simulink model "arducopter"  (R2024b)
settings: Solver=FixedStepAuto  StartTime=0.0  StopTime=simIn.param.timeEnd  FixedStep=simIn.param.dt  RelTol=1e-3
undefined symbols (not defined in the file or in its folder): DiscIntNeverNeededParam, sim, simIn
libraries: simulink x60, slident x4, vrlib x1
(part 7 of 9)

== system arducopter/Attitude Controller/input_euler_angle_roll_pitch_euler_rate_yaw()/Feedforward enabled/input shaping/input shaping yaw rate ==
  note: AC_AttitudeControl::input_shaping_ang_vel()
      | Limits the maximum acceleration resulting from the target yaw rate, so that the target yaw rate is slewed towards the input rate
  yawRateDes : Inport
  yawRateTar : Inport  Port=2
  eulerAccelMax : Inport  Port=3
  Constant2 : Constant  Value=simIn.param.dt  VectorParams1D=off
  Constant3 : Constant  Value=simIn.param.PILOT_Y_RATE_TC  VectorParams1D=off
  Data Type Conversion1 : DataTypeConversion  OutDataTypeStr=single  SaturateOnIntegerOverflow=off  RndMeth=Floor
  MATLAB Function1 : MATLAB Function  TreatAsAtomicUnit=on
  Square Root Controller : Subsystem  TreatAsAtomicUnit=on
  eulerYawRateTar : Outport
  wires:
  yawRateDes/1 -> MATLAB Function1/1(desiredAngVel)
  eulerAccelMax/1 -> MATLAB Function1/3(accelMax)
  MATLAB Function1/1(eulerRateTar) -> eulerYawRateTar/1
  yawRateTar/1 -> MATLAB Function1/2(targetAngVel)
  Data Type Conversion1/1 -> MATLAB Function1/4(dt)
  Constant2/1 -> Data Type Conversion1/1
  Constant3/1 -> MATLAB Function1/5(input_tc)

== system arducopter/Attitude Controller/input_euler_angle_roll_pitch_euler_rate_yaw()/thrust_heading_rotation_angles()/Yaw error limitation/Second limiting condition  ==
  note: Output adapted attitudeTarget and attitudeError if yaw limiting condition is met. Otherwise output old values.
  note: Second limiting condition: if (!is_zero(_p_angle_yaw.kP()) && fabsf(attitude_error.z) > heading_error_max)
  attitudeErrorIn : Inport
  attitudeTargetIn : Inport  Port=2
  thrustVecCorrection : Inport  Port=3
  attitudeBody : Inport  Port=4
  Enable : EnablePort
  Abs : Abs  SaturateOnIntegerOverflow=off
  Compare To Zero : simulink/Logic and Bit Operations/Compare To Zero  relop=~=  OutDataTypeStr=boolean
  Constant3 : Constant  Value=simIn.param.ATC.ACCEL_Y_CONTROLLER_MAX_RADSS
  Constant4 : Constant  Value=simIn.param.ATC.ACCEL_Y_CONTROLLER_MIN_RADSS
  Constant5 : Constant  Value=1/simIn.param.PIDY.P
  Constant6 : Constant  Value=simIn.param.ATC.ACCEL_Y_MAX
  Constant7 : Constant  Value=simIn.param.ATC.ANG_YAW_P
  Constant8 : Constant  Value=simIn.param.ATC.YAW_MAX_ERROR_ANGLE
  Gain1 : Gain  Gain=0.5
  Inverse Square Root Controller : MATLAB Function  TreatAsAtomicUnit=on
  Logical Operator : Logic  AllPortsSameDT=off  OutDataTypeStr=boolean
  Max : MinMax  Function=max  Inputs=2
  Min : MinMax  Inputs=2
  Min1 : MinMax  Inputs=2
  Relational Operator : RelationalOperator  Operator=>  OutDataTypeStr=boolean  RndMeth=Simplest  InputSameDT=off
  Selector2 : Selector  InputPortWidth=3  IndexOptions=Index vector (dialog)  Indices=[3]  OutputSizes=1
  Switch : Switch  Criteria=u2 > Threshold  SaturateOnIntegerOverflow=off  InputSameDT=off
  Switch1 : Switch  Criteria=u2 > Threshold  SaturateOnIntegerOverflow=off  InputSameDT=off
  Yaw limiting and recalculation of attitudeTarget : Subsystem
  attitudeTarget : Outport
  attitudeError : Outport  Port=2
  wires:
  attitudeErrorIn/1 -> [attitudeError]
  Max/1 -> Min/1
  Gain1/1 -> Max/1
  Constant3/1 -> Min/2
  Constant6/1 -> Gain1/1
  Constant4/1 -> Max/2
  Constant5/1 -> Inverse Square Root Controller/1(output)
  Constant7/1 -> Compare To Zero/1, Inverse Square Root Controller/2(p)
  Min/1 -> Inverse Square Root Controller/3(D_max)  "heading_accel_max"
  Constant8/1 -> Min1/2
  Inverse Square Root Controller/1(error) -> Min1/1
  Min1/1 -> Yaw limiting and recalculation of attitudeTarget/2(heading_error_max), Relational Operator/2  "heading_error_max"
  [attitudeError] -> Selector2/1
  Selector2/1 -> Abs/1
  Relational Operator/1 -> Logical Operator/2
  Compare To Zero/1 -> Logical Operator/1
  Abs/1 -> Relational Operator/1
  [attitudeError] -> Switch1/3
  Switch1/1 -> attitudeError/1
  Yaw limiting and recalculation of attitudeTarget/1(attitudeTarget) -> Switch/1
  [attitudeTarget] -> Switch/3
  Yaw limiting and recalculation of attitudeTarget/2(attitudeError) -> Switch1/1
  Switch/1 -> attitudeTarget/1
  Logical Operator/1 -> Yaw limiting and recalculation of attitudeTarget/Enable, Switch1/2, Switch/2
  attitudeBody/1 -> Yaw limiting and recalculation of attitudeTarget/4(attitudeBody)
  thrustVecCorrection/1 -> Yaw limiting and recalculation of attitudeTarget/3(thrustVecCorrection)
  [attitudeError] -> Yaw limiting and recalculation of attitudeTarget/1(attitudeErrorIn)
  attitudeTargetIn/1 -> [attitudeTarget]

== system arducopter/Attitude Controller/input_euler_angle_roll_pitch_euler_rate_yaw()/Feedforward enabled/input shaping/input shaping pitch angle/Square Root Controller1 ==
  sqrt_controller : TriggerPort  TriggerType=function-call  IsSimulinkFunction=on  FunctionName=sqrt_controller  FunctionVisibility=scoped  VariantControl=(inherit)
  Square Root Controller : MATLAB Function  TreatAsAtomicUnit=on
  output : ArgIn  DisableCoverage=on  OutDataTypeStr=single  ArgumentName=err
  p : ArgIn  DisableCoverage=on  Port=2  OutDataTypeStr=single  ArgumentName=p
  D_max : ArgIn  DisableCoverage=on  Port=3  OutDataTypeStr=single  ArgumentName=second_ord_lim
  output1 : ArgIn  DisableCoverage=on  Port=4  OutDataTypeStr=single  ArgumentName=dt
  correctionRate : ArgOut  DisableCoverage=on  OutDataTypeStr=single  ArgumentName=correctionRate
  wires:
  output/1 -> Square Root Controller/1(err)
  p/1 -> Square Root Controller/2(p)
  D_max/1 -> Square Root Controller/3(second_ord_lim)
  Square Root Controller/1(correction_rate) -> correctionRate/1
  output1/1 -> Square Root Controller/4(dt)

== system arducopter/Attitude Controller/input_euler_angle_roll_pitch_euler_rate_yaw()/Feedforward enabled/input shaping/input shaping pitch angle/calc p from input_tc ==
  note: Calculation of proportional factor of square root controller.
      | Based on function argument of sqrt_controller() in AC_AttitudeControl::input_shaping_angle()
  input_tc : Inport
  Constant2 : Constant  Value=0.01  OutDataTypeStr=single
  Constant3 : Constant  OutDataTypeStr=single
  Divide : Product  Inputs=*/
  Max : MinMax  Function=max  Inputs=2
  p : Outport
  wires:
  Constant2/1 -> Max/2
  Max/1 -> Divide/2
  Constant3/1 -> Divide/1
  input_tc/1 -> Max/1
  Divide/1 -> p/1

== system arducopter/Attitude Controller/input_euler_angle_roll_pitch_euler_rate_yaw()/Feedforward enabled/input shaping/input shaping roll angle/Square Root Controller1 ==
  sqrt_controller : TriggerPort  TriggerType=function-call  IsSimulinkFunction=on  FunctionName=sqrt_controller  FunctionVisibility=scoped  VariantControl=(inherit)
  Square Root Controller : MATLAB Function  TreatAsAtomicUnit=on
  output : ArgIn  DisableCoverage=on  OutDataTypeStr=single  ArgumentName=err
  p : ArgIn  DisableCoverage=on  Port=2  OutDataTypeStr=single  ArgumentName=p
  D_max : ArgIn  DisableCoverage=on  Port=3  OutDataTypeStr=single  ArgumentName=second_ord_lim
  output1 : ArgIn  DisableCoverage=on  Port=4  OutDataTypeStr=single  ArgumentName=dt
  correctionRate : ArgOut  DisableCoverage=on  OutDataTypeStr=single  ArgumentName=correctionRate
  wires:
  output/1 -> Square Root Controller/1(err)
  p/1 -> Square Root Controller/2(p)
  D_max/1 -> Square Root Controller/3(second_ord_lim)
  Square Root Controller/1(correction_rate) -> correctionRate/1
  output1/1 -> Square Root Controller/4(dt)

== system arducopter/Attitude Controller/input_euler_angle_roll_pitch_euler_rate_yaw()/Feedforward enabled/input shaping/input shaping roll angle/calc p from input_tc ==
  note: Calculation of proportional factor of square root controller.
      | Based on function argument of sqrt_controller() in AC_AttitudeControl::input_shaping_angle()
  input_tc : Inport
  Constant2 : Constant  Value=0.01  OutDataTypeStr=single
  Constant3 : Constant  OutDataTypeStr=single
  Divide : Product  Inputs=*/
  Max : MinMax  Function=max  Inputs=2
  p : Outport
  wires:
  Constant2/1 -> Max/2
  Max/1 -> Divide/2
  Constant3/1 -> Divide/1
  input_tc/1 -> Max/1
  Divide/1 -> p/1

== system arducopter/Attitude Controller/input_euler_angle_roll_pitch_euler_rate_yaw()/Feedforward enabled/input shaping/input shaping yaw rate/Square Root Controller ==
  sqrt_controller : TriggerPort  TriggerType=function-call  IsSimulinkFunction=on  FunctionName=sqrt_controller  FunctionVisibility=scoped  VariantControl=(inherit)
  Square Root Controller : MATLAB Function  TreatAsAtomicUnit=on
  output : ArgIn  DisableCoverage=on  OutDataTypeStr=single  ArgumentName=err
  p : ArgIn  DisableCoverage=on  Port=2  OutDataTypeStr=single  ArgumentName=p
  D_max : ArgIn  DisableCoverage=on  Port=3  OutDataTypeStr=single  ArgumentName=second_ord_lim
  output1 : ArgIn  DisableCoverage=on  Port=4  OutDataTypeStr=single  ArgumentName=dt
  correctionRate : ArgOut  DisableCoverage=on  OutDataTypeStr=single  ArgumentName=correctionRate
  wires:
  output/1 -> Square Root Controller/1(err)
  p/1 -> Square Root Controller/2(p)
  D_max/1 -> Square Root Controller/3(second_ord_lim)
  Square Root Controller/1(correction_rate) -> correctionRate/1
  output1/1 -> Square Root Controller/4(dt)

== system arducopter/Attitude Controller/input_euler_angle_roll_pitch_euler_rate_yaw()/thrust_heading_rotation_angles()/Yaw error limitation/Second limiting condition /Yaw limiting and recalculation of attitudeTarget ==
  note: Limitation of yaw error
  note: Create new attitudeError with limited yaw error
  note: Calculate new attitudeTarget with limited headingVecCorrection
  attitudeErrorIn : Inport
  heading_error_max : Inport  Port=2
  thrustVecCorrection : Inport  Port=3
  attitudeBody : Inport  Port=4
  Enable : EnablePort
  Constant2 : Constant  Value=0  OutDataTypeStr=single
  Demux : Demux  Outputs=2
  Gain : Gain  Gain=-1
  MATLAB Function1 : MATLAB Function  TreatAsAtomicUnit=on
  MATLAB Function2 : MATLAB Function  TreatAsAtomicUnit=on
  MATLAB Function5 : MATLAB Function  TreatAsAtomicUnit=on
  MATLAB Function9 : MATLAB Function  TreatAsAtomicUnit=on
  Max : MinMax  Function=max  Inputs=2
  Min : MinMax  Inputs=2
  Mux : Mux  Inputs=3
  Mux1 : Mux  Inputs=3
  Selector : Selector  InputPortWidth=3  IndexOptions=Index vector (dialog)  Indices=[3]  OutputSizes=1
  Selector1 : Selector  InputPortWidth=3  IndexOptions=Index vector (dialog)  Indices=[1 2]  OutputSizes=1
  attitudeTarget : Outport
  attitudeError : Outport  Port=2
  wires:
  attitudeErrorIn/1 -> [attitudeError]
  Mux/1 -> MATLAB Function5/1(vec)
  MATLAB Function1/1(qRes) -> attitudeTarget/1
  MATLAB Function9/1(qRes) -> MATLAB Function1/2(q2)
  Min/1 -> Mux1/3, Mux/3
  Mux1/1 -> attitudeError/1
  Selector1/1 -> Demux/1
  Constant2/1 -> Mux/2, Mux/1
  [attitudeError] -> Selector1/1
  attitudeBody/1 -> MATLAB Function1/1(q1)
  Demux/2 -> Mux1/2
  Demux/1 -> Mux1/1
  thrustVecCorrection/1 -> MATLAB Function9/1(q1)
  MATLAB Function5/1(q) -> MATLAB Function9/2(q2)  "headingVecCorrection"
  heading_error_max/1 -> Min/2, Gain/1
  [attitudeError] -> Selector/1
  Gain/1 -> Max/2
  MATLAB Function2/1(radLim) -> Max/1
  Max/1 -> Min/1
  Selector/1 -> MATLAB Function2/1(radIn)

== matlab function arducopter/Position Controller/set_pos_target_z_from_climb_rate()/input_vel_accel_z/MATLAB Function ==
  data: overspeedGain output; velMaxUp input; velMaxDn input; velDes input; overspeedGainDefault input
function overspeedGain = calcOverspeedGain(velMaxUp, velMaxDn, velDes, overspeedGainDefault)
% Calculate increased maximum acceleration and jerk if over speed condition
% is detected
% Code based on AC_PosControl::calculate_overspeed_gain()
overspeedGain = single(1);
if velDes < velMaxDn && velMaxDn ~= 0
    overspeedGain = overspeedGainDefault * velDes / velMaxDn;
end
if velDes > velMaxUp && velMaxUp ~= 0
    overspeedGain = overspeedGainDefault * velDes / velMaxUp;
end

== matlab function arducopter/Position Controller/set_pos_target_z_from_climb_rate()/input_vel_accel_z/update_pos_vel_accel/MATLAB Function ==
  data: posIn input; pos output; velIn input; accIn input; dt input; limit input; vel output; posErr input; velErr input
function [pos, vel] = updatePosVelAccel(posIn, velIn, accIn, dt, limit, posErr, velErr)
% Single axis projection of position and velocity forwards in time based on
% a time step of dt and acceleration off acc.
% Based on update_pos_vel_accel() in control.cpp

% Move position and velocity forward by dt if it does not increase error
% when limited
deltaPos = velIn * dt + accIn * 0.5 * dt^2;
% do not add delta_pos if it will increase the velocity error in the direction of limit
if ((deltaPos * limit) > 0 && (posErr * limit) > 0)
    deltaPos = single(0);
end

pos = posIn + deltaPos;

% The next lines are based on update_vel_accel() which is called from
% update_pos_vel_accel()
deltaVel = accIn * dt;
% do not add delta_vel if it will increase the velocity error in the direction of limit
if ((deltaVel * limit) > 0 && (velErr * limit) > 0)
    if ((velIn * limit) < 0)
        deltaVel = min(max(deltaVel, -abs(velIn)), abs(velIn));
    else
        deltaVel = single(0);
    end
end
vel = velIn + deltaVel;

== matlab function arducopter/Position Controller/set z component of limit vec/MATLAB Function ==
  data: limLower input; limVecZ output; limUpper input
function limVecZ = fcn(limLower, limUpper)
% Based on AC_PosControl::update_z_controller()

if limUpper
    limVecZ = single(1);
elseif limLower
    limVecZ = single(-1);
else
    limVecZ = single(0);
end

== matlab function arducopter/Position Controller/set_pos_target_z_from_climb_rate()/input_vel_accel_z/shape_vel_accel/calc_KPa ==
  data: velErr output; velIn input; KPa output; vel input; accMin input; accMax input; jerkMax input
function [velErr, KPa] = calcKPa(velIn, vel, accMin, accMax, jerkMax)
% First part of shape_vel_accel() in control.cpp
% Calculates correction gain KPa for the square root controller based on
% the jerk and acceleration limits.

% Velocity error to be corrected
velErr = velIn - vel;

% Calculate time constants and limits to ensure stable operation.
% The direction of acceleration limit is the same as the velocity error.
% This is because the velocity error is negative when slowing down while
% closing a positive position error.
if velErr > 0
    KPa = jerkMax / accMax;
else
    KPa = jerkMax / (-accMin);
end

== matlab function arducopter/Position Controller/set_pos_target_z_from_climb_rate()/input_vel_accel_z/shape_vel_accel/Square Root Controller ==
  data: err input; correction_rate output; p input; second_ord_lim input; dt input
function correction_rate = sqrt_controller(err, p, second_ord_lim, dt)
% The square root controller
% Code is taken from sqrt_controller(...) in AC_PosControl.cpp.

if (second_ord_lim < 0 || second_ord_lim == 0)
   correction_rate = err * p;
elseif (p == 0)
    % P term is zero, but second order limit is positive
    if (err > 0)
        correction_rate = sqrt(single(2.0) * second_ord_lim * err);
    elseif (err < 0)
        correction_rate = sqrt(single(2.0) * second_ord_lim * -err);
    else
        correction_rate = single(0.0);
    end
else
    % P term and second order limit are positive, hence have been defined
    linear_dist = second_ord_lim / (p * p);
    % Check if error exceeds linear range of controller gain
    if (err > linear_dist)
        correction_rate = sqrt(single(2.0) * second_ord_lim * ( err - (linear_dist / single(2.0)) ));
    elseif (err < -linear_dist)
        correction_rate = -sqrt(single(2.0) * second_ord_lim * ( -err - (linear_dist / single(2.0)) ));
    else
        % Return linearly amplified correction if error is in linear range
        correction_rate = err * p;
    end
end

% Prevent oscillations by over-shooting the error correction in the last
% time step
if (dt > 0)
    correction_rate = min( max(correction_rate, -abs(err) / dt), abs(err) / dt);
end

== matlab function arducopter/Position Controller/set_pos_target_z_from_climb_rate()/input_vel_accel_z/shape_vel_accel/MATLAB Function ==
  data: accTar input; accShaped output; accMin input; accMax input; accIn input; acc input; jerkMax input; dt input; limitTotalAccel input
function accShaped = shapeAccelDes(accTar, accMin, accMax, accIn, acc, jerkMax, dt, limitTotalAccel)
% Second part of shape_vel_accel() in control.cpp
% Constrains desired acceleration based on acceleration limits and shapes
% kinematic path according to max jerk

%% 1) Limit desired acceleration based on acceleration limits
% Constrain correction acceleration from accMin to accMax
accTar = max(min(accTar, accMax), accMin);

% Velocity correction with input velocity
accTar = accTar + accIn;

% Constrain total acceleration from accMin to accMax
if limitTotalAccel
    accTar = max(min(accTar, accMax), accMin);
end

%% 2) Calculate required jerk limited adjustment to the current acceleration
% for the next time dt. Based on shape_accel()
accShaped = acc;
if (dt > 0)
    accDelta = accTar - acc;
    accDelta = min(max(accDelta, -jerkMax * dt), jerkMax * dt);
    accShaped = acc + accDelta;
end

== matlab function arducopter/Throttle/Throttle Calculations/Throttle Hover/Throttle Hover Calculation ==
  data: thrHover output single; dt input; thrAct input; zVelDes input; zVelAct input; thstHoverMax input; thstHoverMin input; thstHoverTC input; thstHoverDefault input; hoverLearn input; thrMan input; thrHoverAct data_store_memory
function thrHover = updateThrHov(dt, thrAct, zVelDes, zVelAct, thstHoverMax, thstHoverMin, thstHoverTC, thstHoverDefault, hoverLearn, thrMan)
%% Code is based on Copter::update_throttle_hover() in Attitude.cpp

global thrHoverAct;

% Use default throttle hover when throttle is set to manual
if (thrMan)
    thrHover = thrHoverAct;
    return;
    % thrHoverAct = thstHoverDefault;
end
if zVelDes > 0
    thrHover = thrHoverAct;
    return;
    % thrHoverAct = thstHoverDefault;
end


% Calc average throttle if we are in level hover
if (thrAct > 0  && abs(zVelAct) < 60)
    %% Code is based on AP_MotorsMulticopter::update_throttle_hover(dt) in AP_MotorsMulticopter.cpp
    % Update throttle hover in dependency of the current output throttle
    if ( (hoverLearn ~= 0))
        thrHoverAct = thrHoverAct + (dt / (dt + thstHoverTC) ) * (thrAct - thrHoverAct);

        % Limit throttle hover to specified limits
        thrHoverAct = min( max( thrHoverAct, thstHoverMin), thstHoverMax);
    end
end

thrHover = thrHoverAct;

== matlab function arducopter/Position Controller/get_pilot_speed_dn()/MATLAB Function ==
  data: dnMaxIn input; dnMax output; upMax input
function dnMax = getPilotSpeedDown(dnMaxIn, upMax)
% Get maximum vertical descending velocity. Called in ModeAltHold::init()
% in the function call for AC_PosControl::set_max_speed_accel_z()
if dnMaxIn == 0
    dnMax = abs(upMax);
else
    dnMax = abs(dnMaxIn);
end

== matlab function arducopter/Attitude Controller/input_euler_angle_roll_pitch_euler_rate_yaw()/Feedforward enabled/input shaping/input shaping pitch angle/Square Root Controller1/Square Root Controller ==
  data: err input; correction_rate output; p input; second_ord_lim input; dt input
function correction_rate = sqrt_controller(err, p, second_ord_lim, dt)
% The square root controller
% Code is taken from sqrt_controller(...) in AC_PosControl.cpp.

if (second_ord_lim < 0 || second_ord_lim == 0)
   correction_rate = err * p;
elseif (p == 0)
    % P term is zero, but second order limit is positive
    if (err > 0)
        correction_rate = sqrt(single(2.0) * second_ord_lim * err);
    elseif (err < 0)
        correction_rate = sqrt(single(2.0) * second_ord_lim * -err);
    else
        correction_rate = single(0.0);
    end
else
    % P term and second order limit are positive, hence have been defined
    linear_dist = second_ord_lim / (p * p);
    % Check if error exceeds linear range of controller gain
    if (err > linear_dist)
        correction_rate = sqrt(single(2.0) * second_ord_lim * ( err - (linear_dist / single(2.0)) ));
    elseif (err < -linear_dist)
        correction_rate = -sqrt(single(2.0) * second_ord_lim * ( -err - (linear_dist / single(2.0)) ));
    else
        % Return linearly amplified correction if error is in linear range
        correction_rate = err * p;
    end
end

% Prevent oscillations by over-shooting the error correction in the last
% time step
if (dt ~= 0)
    correction_rate = max( min(correction_rate, abs(err) / dt), -abs(err) / dt);
end

== matlab function arducopter/Attitude Controller/input_euler_angle_roll_pitch_euler_rate_yaw()/Feedforward enabled/input shaping/input shaping roll angle/Square Root Controller1/Square Root Controller ==
  data: err input; correction_rate output; p input; second_ord_lim input; dt input
function correction_rate = sqrt_controller(err, p, second_ord_lim, dt)
% The square root controller
% Code is taken from sqrt_controller(...) in AC_PosControl.cpp.

if (second_ord_lim < 0 || second_ord_lim == 0)
   correction_rate = err * p;
elseif (p == 0)
    % P term is zero, but second order limit is positive
    if (err > 0)
        correction_rate = sqrt(single(2.0) * second_ord_lim * err);
    elseif (err < 0)
        correction_rate = sqrt(single(2.0) * second_ord_lim * -err);
    else
        correction_rate = single(0.0);
    end
else
    % P term and second order limit are positive, hence have been defined
    linear_dist = second_ord_lim / (p * p);
    % Check if error exceeds linear range of controller gain
    if (err > linear_dist)
        correction_rate = sqrt(single(2.0) * second_ord_lim * ( err - (linear_dist / single(2.0)) ));
    elseif (err < -linear_dist)
        correction_rate = -sqrt(single(2.0) * second_ord_lim * ( -err - (linear_dist / single(2.0)) ));
    else
        % Return linearly amplified correction if error is in linear range
        correction_rate = err * p;
    end
end

% Prevent oscillations by over-shooting the error correction in the last
% time step
if (dt ~= 0)
    correction_rate = max( min(correction_rate, abs(err) / dt), -abs(err) / dt);
end

== matlab function arducopter/Attitude Controller/input_euler_angle_roll_pitch_euler_rate_yaw()/Feedforward enabled/input shaping/input shaping yaw rate/Square Root Controller/Square Root Controller ==
  data: err input; correction_rate output; p input; second_ord_lim input; dt input
function correction_rate = sqrt_controller(err, p, second_ord_lim, dt)
% The square root controller
% Code is taken from sqrt_controller(...) in AC_PosControl.cpp.

if (second_ord_lim < 0 || second_ord_lim == 0)
   correction_rate = err * p;
elseif (p == 0)
    % P term is zero, but second order limit is positive
    if (err > 0)
        correction_rate = sqrt(single(2.0) * second_ord_lim * err);
    elseif (err < 0)
        correction_rate = sqrt(single(2.0) * second_ord_lim * -err);
    else
        correction_rate = single(0.0);
    end
else
    % P term and second order limit are positive, hence have been defined
    linear_dist = second_ord_lim / (p * p);
    % Check if error exceeds linear range of controller gain
    if (err > linear_dist)
        correction_rate = sqrt(single(2.0) * second_ord_lim * ( err - (linear_dist / single(2.0)) ));
    elseif (err < -linear_dist)
        correction_rate = -sqrt(single(2.0) * second_ord_lim * ( -err - (linear_dist / single(2.0)) ));
    else
        % Return linearly amplified correction if error is in linear range
        correction_rate = err * p;
    end
end

% Prevent oscillations by over-shooting the error correction in the last
% time step
if (dt ~= 0)
    correction_rate = max( min(correction_rate, abs(err) / dt), -abs(err) / dt);
end

== matlab function arducopter/Throttle/Throttle Calculations/Throttle-Attitude-Mixing/get_throttle_hover/MATLAB Function ==
  data: thrHover input; thrHoverLim output; thrHoverMin input; thrHoverMax input
function thrHoverLim = constrain(thrHover, thrHoverMin, thrHoverMax)

thrHoverLim = min( max( thrHover, thrHoverMin), thrHoverMax);

== matlab function arducopter/Attitude Controller/Determine angleLimit/MATLAB Function2 ==
  data: altholdLeanAngleMax input; altholdLeanAngleMaxCDeg output; angleLimitMin input
function altholdLeanAngleMaxCDeg = get_althold_lean_angle_max_cd(altholdLeanAngleMax, angleLimitMin)
% Based on AC_AttitudeControl::get_althold_lean_angle_max_cd().
% Function calculates a tilt angle limit for pilot input that prioritises
% altitude hold over lean angle.
altholdLeanAngleMaxCDeg = max(180/pi * altholdLeanAngleMax, angleLimitMin) * 100;

== matlab function arducopter/Throttle/Throttle Calculations/MATLAB Function ==
  data: thrThstMax input; throttle_in input; angleLimitTc input; dt input; angleLimitThrMax input; altholdLeanAngleMax_ data_store_memory; altholdLeanAngleMax output
function altholdLeanAngleMax = update_althold_lean_angle_max(thrThstMax, throttle_in, angleLimitTc, dt, angleLimitThrMax)
% Based on AC_AttitudeControl_Multi::update_althold_lean_angle_max. 
% Function updates Althold angle maximum.

global altholdLeanAngleMax_

if thrThstMax == 0
    altholdLeanAngleMax_ = single(0);
    altholdLeanAngleMax = single(0);
    return;
end

altholdLeanAngleMax = acos(min(max(throttle_in / (angleLimitThrMax * thrThstMax), single(0)), single(1)));
altholdLeanAngleMax_ = altholdLeanAngleMax_ + (dt / (dt + angleLimitTc)) * (altholdLeanAngleMax - altholdLeanAngleMax_);
altholdLeanAngleMax = altholdLeanAngleMax_;

== matlab function arducopter/Attitude Controller/input_euler_angle_roll_pitch_euler_rate_yaw()/thrust_heading_rotation_angles()/Yaw error limitation/Second limiting condition /Inverse Square Root Controller ==
  data: output input; error output; p input; D_max input
function error = inv_sqrt_controller(output, p, D_max)
% The inverse square root controller
% inv_sqrt_controller calculates the inverse of the sqrt controller.
% This function calculates the input (aka error) to the sqrt_controller required to achieve a given output.
% Code is taken from inv_sqrt_controller(...) in AP_Math\control.cpp


if (D_max > 0 && p == 0)
    error = (output * output) / (2 * D_max);
    return;
end

if (D_max <= 0 && p ~= 0)
    error = output / p;
    return;
end

if (D_max <= 0 && p ~= 0)
    error = single(0);
    return;
end

% calculate the velocity at which we switch from calculating the stopping point using a linear function to a sqrt function.
linear_velocity = D_max / p;

if (abs(output) < linear_velocity) 
    % if our current velocity is below the cross-over point we use a linear function
    error = output / p;
    return;
end

linear_dist = D_max / (p * p);
stopping_dist = (linear_dist * 0.5) + (output * output) / (2 * D_max);
if (output > 0)
    error = stopping_dist;
else
    error = -stopping_dist;
end

== matlab function arducopter/Rate Controller/PID Yaw Rate/Slew Limiter/Lowpass Filter ==
  data: in input; out output single; alpha input; out_last input
function out  = apply(in, alpha, out_last)
% The code is based on the apply(sample, cutoff_freq, dt) function in
% LowPassFilter.cpp

% Output calculation
out = out_last + (in - out_last) * alpha;

== matlab function arducopter/Attitude Controller/input_euler_angle_roll_pitch_euler_rate_yaw()/thrust_heading_rotation_angles()/Yaw error limitation/Second limiting condition /Yaw limiting and recalculation of attitudeTarget/MATLAB Function2 ==
  data: radIn input; radLim output
function radLim = wrapPi(radIn)
% Function to limit input angle in radian to [-pi pi].
% Code based on wrap_PI() and wrap_2PI() of AP_Math.cpp

% 1) Limit to [0 2pi]
radLim = mod(radIn, 2*pi);
if radLim < 0
    radLim = radLim + 2*pi;
end

% 2) Limit to [0 pi]
if radLim > pi
    radLim = radLim - 2*pi;
end

== matlab function arducopter/Attitude Controller/input_euler_angle_roll_pitch_euler_rate_yaw()/thrust_heading_rotation_angles()/Yaw error limitation/Second limiting condition /Yaw limiting and recalculation of attitudeTarget/MATLAB Function1 ==
  data: q1 input; qRes output; q2 input
function qRes = quatMult(q1, q2)
% Quaternion multiplication. Code based on QuaternionT<T>::operator*() in
% quaternion.cpp

qRes = single(zeros(4,1));
qRes(1) = q1(1)*q2(1) - q1(2)*q2(2) - q1(3)*q2(3) - q1(4)*q2(4);
qRes(2) = q1(1)*q2(2) + q1(2)*q2(1) + q1(3)*q2(4) - q1(4)*q2(3);
qRes(3) = q1(1)*q2(3) - q1(2)*q2(4) + q1(3)*q2(1) + q1(4)*q2(2);
qRes(4) = q1(1)*q2(4) + q1(2)*q2(3) - q1(3)*q2(2) + q1(4)*q2(1);

== matlab function arducopter/Attitude Controller/input_euler_angle_roll_pitch_euler_rate_yaw()/thrust_heading_rotation_angles()/Yaw error limitation/Second limiting condition /Yaw limiting and recalculation of attitudeTarget/MATLAB Function5 ==
  data: vec input; q output
function q = fromAxisAngle(vec)
% Create a quaternion from its axis-angle representation. Just the rotation
% vector is given as input.
% Based on QuaternionT<T>::from_axis_angle(Vector3<T>)

q = single(zeros(4,1));
angle = sqrt(vec(1)^2 + vec(2)^2 + vec(3)^2);

if angle == 0
    q(1) = 1;
    q(2) = 0;
    q(3) = 0;
    q(4) = 0;
else
    axis = vec ./ angle;
    % The following lines are based on QuaternionT<T>::from_axis_angle(const Vector3<T> &axis, T theta)
    if angle == 0
        q(1) = 1;
        q(2) = 0;
        q(3) = 0;
        q(4) = 0;
    else
        st2 = sin(0.5*angle);
        q(1) = cos(0.5*angle);
        q(2) = axis(1) * st2;
        q(3) = axis(2) * st2;
        q(4) = axis(3) * st2;
    end
end

== matlab function arducopter/Attitude Controller/input_euler_angle_roll_pitch_euler_rate_yaw()/thrust_heading_rotation_angles()/Yaw error limitation/Second limiting condition /Yaw limiting and recalculation of attitudeTarget/MATLAB Function9 ==
  data: q1 input; qRes output; q2 input
function qRes = quatMult(q1, q2)
% Quaternion multiplication. Code based on QuaternionT<T>::operator*() in
% quaternion.cpp

qRes = single(zeros(4,1));
qRes(1) = q1(1)*q2(1) - q1(2)*q2(2) - q1(3)*q2(3) - q1(4)*q2(4);
qRes(2) = q1(1)*q2(2) + q1(2)*q2(1) + q1(3)*q2(4) - q1(4)*q2(3);
qRes(3) = q1(1)*q2(3) - q1(2)*q2(4) + q1(3)*q2(1) + q1(4)*q2(2);
qRes(4) = q1(1)*q2(4) + q1(2)*q2(3) - q1(3)*q2(2) + q1(4)*q2(1);

== matlab function arducopter/Throttle/Throttle Calculations/Throttle Limiting based on battery state/Update Lift Max from Battery Voltage ==
  data: battVoltFiltLast input; battVoltFilt output single; battVoltRestEst input; liftMax output single; battVoltMax input; battVoltMin input single; thstCurveExpo input; battVoltMinAct output single; battVoltRestEstAct output single; loop_rate input
function [battVoltFilt, liftMax, battVoltMinAct, battVoltRestEstAct] = update_lift_max_from_batt_voltage(battVoltFiltLast, battVoltRestEst, battVoltMax, battVoltMin, thstCurveExpo, loop_rate)
% Code taken from AP_MotorsMulticopter::update_lift_max_from_batt_voltage()
% in AP_MotorsMulticopter.cpp

% new 4.6.2 in Thrust_Linearization::update_lift_max_from_batt_voltage()
% TODO: make optrion BATT_RAW_VOLTAGE == 0 possible

% Check if batt_volt_min is too small
if (battVoltMax <= 0 || (battVoltMin >= battVoltMax) ...
        || battVoltRestEst < 0.25 * battVoltMin)
    battVoltFilt = single(1.0);
    liftMax = single(1.0);
    battVoltMinAct = battVoltMin;
    battVoltRestEstAct = battVoltRestEst;
    return;
end

% Set lower battery voltage limit for thrust scaling to a new value
battVoltMinAct = max(battVoltMin, battVoltMax * 0.6);

% Constrain resting voltage estimate (resting voltage is actual voltage
% with sag removed based on current draw and resistance)
battVoltRestEstAct = min( max(battVoltRestEst, battVoltMin), battVoltMax);

%% Filter battery voltage at 0.5 Hz. 
% Cutoff Frequency defined in AP_MotorsMulticopter.h
cutoff_freq = single(0.5);
% Calculate time constant and alpha value
T = 1 / (2 * pi * cutoff_freq);
dt = 1 / loop_rate;
alpha = dt / (dt + T);
alpha = max( min( alpha, 1.0), 0.0);

% Filter input is batt_volt_rest_est / batt_volt_comp_max
in = battVoltRestEstAct / battVoltMax;

% Output calculation
battVoltFilt = battVoltFiltLast + (in - battVoltFiltLast) * alpha;

%% Calculate lift_max
thstCurveExpo = min( max(thstCurveExpo, -1), 1);
liftMax = battVoltFilt * (1 - thstCurveExpo) + thstCurveExpo * battVoltFilt * battVoltFilt;

== matlab function arducopter/Throttle/Throttle Calculations/Throttle Limiting based on battery state/Get current throttle limit ==
  data: thrThstMax output; batVoltMin input; batCurrMax input; batCurrT input; loop_rate input; batCurr input; batRes input; batVolt input; thrLimit output; thrHover input; thrLimitLast input single
function [thrThstMax, thrLimit] = get_current_limit_max_throttle(batVoltMin, batCurrMax, batCurrT, loop_rate, batCurr, batRes, batVolt, thrHover, thrLimitLast)
% Code is based on AP_MotorsMulticopter::get_current_limit_max_throttle()
% in AP_MotorsMulticopter.cpp. 
% Returns a throttle limit based on the maximum battery current as a number
% from 0~1 in the range throttle_min to throttle_max.

% Return maximum if current limiting is disabled
if(batCurrMax <= 0) 
    thrLimit = single(1.0);
    thrThstMax = single(1.0);
    return;
end
% Return maximum if battery resistance is not measured
if(batRes == 0)
    thrLimit = single(1.0);
    thrThstMax = single(1.0);
    return;
end

%% Calculate throttle limit
% The throttle limit represents the maximum throttle potential that is left
% based on the actual current compared to the maximum battery current.

% Maximum current to prevent voltage sag below batt_voltage_min
% Since the actual battery current level is used as the minimum for the limit,
% the actual current can still be used to maintain the current throttle. 
batt_curr_max_new = min(batCurrMax, batCurr + (batVolt - batVoltMin) / batRes);
% Calcualte current artion
batt_curr_ratio = batCurr / batt_curr_max_new;
% Calculate time step
dt = 1 / loop_rate;
% Calculate throttle limit as the additional throttle on top of throttle
% hover
thrLimit = thrLimitLast + (dt / (dt + batCurrT)) * (1.0 - batt_curr_ratio);
% Throttle limit drops to 20% between hover an full throttle
thrLimit = min( max( thrLimit, 0.2), 1);

% Calculate maximum throttle as sum of hover throttle and the possible
% additional throttle based on the maximum current.
thrThstMax = thrHover + ((1.0 - thrHover) * thrLimit);

== matlab function arducopter/Rate Controller/PID Yaw Rate/I/Integrator ==
  data: error input; integrator_out output; integrator input single; limit_flg input; ki input; i_max input; dt input
function integrator_out = fcn(error, integrator, limit_flg, ki, i_max, dt)
% Code is based on AC_PID::update_i() in AC_PID.cpp.

% Check plausibility of input parameters
if (ki ~= 0 && dt > 0)
    % Only allow integration if limit is not set or the absolute sum of the
    % integrator would be reduced.
    if (~limit_flg || (integrator > 0 && error < 0) || (integrator < 0 && error > 0))
        integrator_out = integrator + error * ki * dt;
        integrator_out = max( min(integrator_out, i_max), -i_max);
    else % Otherwise, keep old integrator value
        integrator_out = integrator;
    end
else % Reset integrator if input parameters are not plausible
    integrator_out = single(0.0);
end

== matlab function arducopter/Rate Controller/PID Roll Rate/I/Integrator ==
  data: error input; integrator_out output; integrator input single; limit_flg input; ki input; i_max input; dt input
function integrator_out = fcn(error, integrator, limit_flg, ki, i_max, dt)
% Code is based on AC_PID::update_i() in AC_PID.cpp.

% Check plausibility of input parameters
if (ki ~= 0 && dt > 0)
    % Only allow integration if limit is not set or the absolute sum of the
    % integrator would be reduced.
    if (~limit_flg || (integrator > 0 && error < 0) || (integrator < 0 && error > 0))
        integrator_out = integrator + error * ki * dt;
        integrator_out = max( min(integrator_out, i_max), -i_max);
    else % Otherwise, keep old integrator value
        integrator_out = integrator;
    end
else % Reset integrator if input parameters are not plausible
    integrator_out = single(0.0);
end

== matlab function arducopter/Throttle/Throttle Calculations/Get compensation gain ==
  data: liftMax input; compGain output single; airDensityRatio input
function compGain = get_compensation_gain(liftMax, airDensityRatio)
% Code is based on AP_MotorsMulticopter::get_compensation_gain() in
% AP_MotorsMulticopter.cpp.

% Avoid to divide by zero
if(liftMax <= 0.0)
    compGain = single(1.0);
    return;
end

compGain = 1.0 / liftMax;

% Limit air density ratio
airDensityRatioLim = double(min( max( airDensityRatio, 0.5 ), 1.25));

if (airDensityRatio > 0.3 && airDensityRatio < 1.5)
   compGain = compGain * (1.0 / airDensityRatioLim); 
end

== matlab function arducopter/Rate Controller/PID Roll Rate/Slew Limiter/Calculate Dmod ==
  data: slew_rate input; Dmod output single; sr_max input; sr_tau input; dt input; time input; pos_event_idx data_store_memory; pos_event_stored data_store_memory; pos_event_ms data_store_memory; neg_event_idx data_store_memory; neg_event_stored data_store_memory; neg_event_ms data_store_memory; modifier_slew_rate data_store_memory; output_slew_rate data_store_memory; max_neg_slew_event_ms data_store_memory; max_pos_slew_event_ms data_store_memory; max_neg_slew_rate data_store_memory; max_pos_slew_rate data_store_memory
function Dmod   = fcn(slew_rate, sr_max, sr_tau, dt, time)
% Code is based on SlewLimiter::modifier() in SlewLimiter.cpp. 

% Define global variables, so that quanitities do not have to be fed back
% to the function
global pos_event_stored;
global pos_event_idx;
global pos_event_ms;
global max_pos_slew_rate;
global max_pos_slew_event_ms;
global neg_event_stored;
global neg_event_idx;
global neg_event_ms;
global max_neg_slew_rate;
global max_neg_slew_event_ms;
global modifier_slew_rate;
global output_slew_rate;

% Definition of constants as done in SlewLimiter.h
SLEWLIMITER_N_EVENTS = uint32(3); % Number of positive and negative consecutive slew rate exceedance events recorded. Set to 3 because of 1-based indexing.
WINDOW_MS = uint32(300); % Time in ms required for half a cycle of the slowest oscillation frequency expected
MODIFIER_GAIN = 1.5; % Ratio of modifier reduction to slew rate exceedance

if (dt < 0)
    Dmod = single(1.0);
    return;
end

now_ms = uint32(time);
decay_alpha = min(dt, sr_tau) / sr_tau;

% Apply a filter to decay maximum seen slew rate once the value had left the window period
attack_alpha = min(2.0 * decay_alpha, 1.0);

%% Calculate maximum slew rate
% Save new maximum slew rates, if oldest maximum is exceeded
% OR decay the peak slew rates (pos. and neg.) if they are outside the
% observed time window
% Never drop PID gains below 10% of configured value
if (slew_rate > max_pos_slew_rate)
    max_pos_slew_rate(:) = slew_rate;
    max_pos_slew_event_ms = now_ms;
elseif (now_ms - max_pos_slew_event_ms > WINDOW_MS)
    max_pos_slew_rate = max_pos_slew_rate * (1.0 - decay_alpha);
end

if (-slew_rate > max_neg_slew_rate)
    max_neg_slew_rate(:) = -slew_rate;
    max_neg_slew_event_ms = now_ms;
elseif (now_ms - max_neg_slew_event_ms > WINDOW_MS)
    max_neg_slew_rate = max_neg_slew_rate * (1.0 - decay_alpha);
end

% Calculate the averaged maximum slew rate
raw_slew_rate = 0.5 * (max_pos_slew_rate + max_neg_slew_rate);
% Calculation of output slew rate
output_slew_rate = output_slew_rate + (raw_slew_rate - output_slew_rate) * attack_alpha;
output_slew_rate = min(raw_slew_rate, output_slew_rate);

% Check if slew limiter is activated
if(sr_max <= 0)
   Dmod = single(1.0);
   return;
end

% Constrain slew rate used for calculation
limited_raw_slew_rate = 0.5 * (min(max_pos_slew_rate, 10 * sr_max) + min(max_neg_slew_rate, 10 * sr_max));


%% Save exceedance events in event time vector
% Store a series of positive slew rate exceedance events
if (~pos_event_stored && slew_rate > sr_max)
    if (pos_event_idx >= SLEWLIMITER_N_EVENTS)
        pos_event_idx(:) = 1;
    end
    pos_event_ms(pos_event_idx) = now_ms;
    pos_event_idx(:) = pos_event_idx + 1;
    pos_event_stored = true;
    neg_event_stored = false;
end

% Store a series of negative slew rate exceedance events
if (~neg_event_stored && -slew_rate > sr_max)
    if (neg_event_idx >= SLEWLIMITER_N_EVENTS)
        neg_event_idx(:) = 1;
    end
    neg_event_ms(neg_event_idx) = now_ms;
    neg_event_idx(:) = neg_event_idx + 1;
    pos_event_stored = false;
    neg_event_stored = true;
end

% Find oldest event time
oldest_ms = now_ms;
for i=1:SLEWLIMITER_N_EVENTS-1
   oldest_ms = min(oldest_ms, pos_event_ms(i));
   oldest_ms = min(oldest_ms, neg_event_ms(i));
end

% When the oldest exceedance event falls outside of the window required for
% the number of exceedance events, apply a further reduction to the maximum
% slew rate. This prevents unwanted gain reductions caused by spikes in the
% demanded angular rates due to changed control modes or similar causes.
modifier_input = limited_raw_slew_rate;
if(now_ms - oldest_ms > SLEWLIMITER_N_EVENTS * WINDOW_MS) % no incrementation of SLEWLIMITER_N_EVENTS because of 1 based indexing
   oldest_time_from_window = single(0.001) * single(now_ms - oldest_ms - SLEWLIMITER_N_EVENTS * WINDOW_MS); 
   modifier_input = modifier_input * single(exp(-oldest_time_from_window / sr_tau));
end

%% Calculation of modifier slew rate

modifier_slew_rate = modifier_slew_rate + (modifier_input - modifier_slew_rate) * attack_alpha;
modifier_slew_rate = min(modifier_slew_rate, modifier_input);

% Calculate modifier. Only has an impact if sr_max is exceeded by averaged
% slew rate.
if(modifier_slew_rate > sr_max)
    Dmod(:) = sr_max / (sr_max + MODIFIER_GAIN * (modifier_slew_rate - sr_max));
else
    Dmod(:) = 1.0;
end

== matlab function arducopter/Rate Controller/PID Roll Rate/Slew Limiter/Lowpass Filter ==
  data: in input; out output single; alpha input; out_last input
function out  = apply(in, alpha, out_last)
% The code is based on the apply(sample, cutoff_freq, dt) function in
% LowPassFilter.cpp

% Output calculation
out = out_last + (in - out_last) * alpha;

== matlab function arducopter/Throttle/Throttle Calculations/Air density Calculation/Get equivalent to true airspeed EAS2TAS ==
  data: alt input; eas2tas output; airPress input; gndTemp input; EAS2TAS data_store_memory; last_alt_EAS2TAS data_store_memory
function eas2tas = fcn(alt, airPress, gndTemp)
% Code is based on AP_Baro::get_EAS2TAS() in AP_Baro.cpp.

% Constants
C_TO_KELVIN = single(273.15); % Conversion offset from celsius to kelvin
ISA_LAPSE_RATE = single(0.0065);
ISA_GAS_CONSTANT = single(287.26);
SSL_AIR_DENSITY = single(1.225);

% Global variables
global EAS2TAS;
global last_alt_EAS2TAS;

% Check if altitude has changed significally
if ((abs(alt - last_alt_EAS2TAS) < 25.0) && EAS2TAS ~= 0)
    % Change too small to require re-calculating
   eas2tas = EAS2TAS;
   return;
end

if (airPress == 0)
   eas2tas = single(1.0);
   return;
end

tempK = single(gndTemp + C_TO_KELVIN - ISA_LAPSE_RATE * alt);
eas2tas_squared = SSL_AIR_DENSITY / (airPress / (ISA_GAS_CONSTANT * tempK));
if (eas2tas_squared <= 0)
    eas2tas = single(1.0);
    return;
end
EAS2TAS = sqrt(eas2tas_squared);
last_alt_EAS2TAS = alt;
eas2tas = EAS2TAS;

== matlab function arducopter/Throttle/Throttle Calculations/Air density Calculation/Get air density ratio ==
  data: eas2tas input; airDensityRatio output
function airDensityRatio = fcn(eas2tas)
% Code is based on AP_Baro::get_air_density_ratio() in AP_Baro.cpp.
if (eas2tas > 0.0)
    airDensityRatio = single(1.0 / (eas2tas*eas2tas));
else
    airDensityRatio = single(1.0);
end

== matlab function arducopter/Attitude Controller/input_euler_angle_roll_pitch_euler_rate_yaw()/Feedforward enabled/input shaping/input shaping pitch angle/MATLAB Function1 ==
  data: desiredAngVel input; targetAngVel input; eulerRateTar output; accelMax input; dt input; input_tc input
function eulerRateTar = input_shaping_ang_vel(desiredAngVel, targetAngVel, accelMax, dt, input_tc)
% Limits acceleration and deceleration of a velocity request
% Code based on AC_AttitudeControl::input_shaping_ang_vel()

if input_tc > 0
    % Calculate the acceleration to smoothly achieve rate. Jerk is not limited.
    errorRate = desiredAngVel - targetAngVel;
    desiredAngAccel = sqrt_controller(errorRate, 1.0/max(input_tc, single(0.01)), single(0), dt);
    desiredAngVel = targetAngVel + desiredAngAccel * dt;
end

% Acceleration is limited directly to smooth the beginning of the curve
if accelMax > 0
    deltaAngVel = accelMax * dt;
    eulerRateTar = min(max(desiredAngVel, targetAngVel - deltaAngVel), targetAngVel + deltaAngVel);
else
    eulerRateTar = desiredAngVel;
end

== matlab function arducopter/Attitude Controller/input_euler_angle_roll_pitch_euler_rate_yaw()/Feedforward enabled/input shaping/input shaping yaw rate/MATLAB Function1 ==
  data: desiredAngVel input; targetAngVel input; eulerRateTar output; accelMax input; dt input; input_tc input
function eulerRateTar = input_shaping_ang_vel(desiredAngVel, targetAngVel, accelMax, dt, input_tc)
% Limits acceleration and deceleration of a velocity request
% Code based on AC_AttitudeControl::input_shaping_ang_vel()

if input_tc > 0
    % Calculate the acceleration to smoothly achieve rate. Jerk is not limited.
    errorRate = desiredAngVel - targetAngVel;
    desiredAngAccel = sqrt_controller(errorRate, 1.0/max(input_tc, single(0.01)), single(0), dt);
    desiredAngVel = targetAngVel + desiredAngAccel * dt;
end

% Acceleration is limited directly to smooth the beginning of the curve
if accelMax > 0
    deltaAngVel = accelMax * dt;
    eulerRateTar = min(max(desiredAngVel, targetAngVel - deltaAngVel), targetAngVel + deltaAngVel);
else
    eulerRateTar = desiredAngVel;
end

== matlab function arducopter/Rate Controller/PID Yaw Rate/MATLAB Function ==
  data: p_in input; p_out output; d_in input; pd_max input; d_out output; boost input
function [p_out, d_out] = pd_sum_limit(p_in, d_in, pd_max, boost)
% Code is based on AC_PID::update_all() in AC_PID.cpp

% Boost output if required
p_out = p_in * boost;
d_out = d_in * boost;

% Apply PD sum limit if enabled
if (pd_max > 0)
    pd_sum = abs(p_in + d_in);
    if (pd_sum > pd_max)
        PD_scale = pd_max / pd_sum;
        p_out = p_in * PD_scale;
        d_out = d_in * PD_scale;
    end
end
